simulink model "Q2_All"  (R2023b)
settings: Solver=VariableStepAuto  StartTime=0.0  StopTime=2000  RelTol=1e-3
libraries: simulink x17
settings Model: Creator=ArshiaGosh  LastModifiedBy=ArshiaGosh

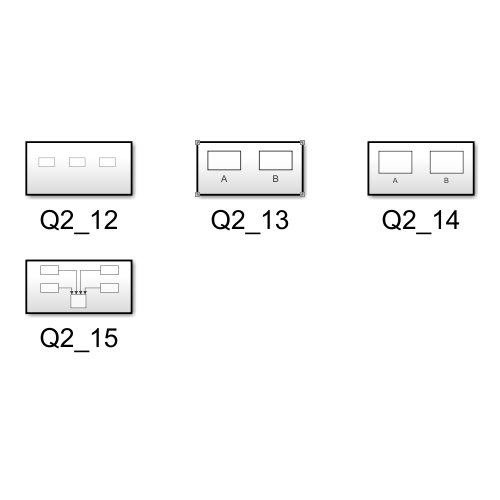
[thumbnail: Simulink's stored preview of the top-level diagram]
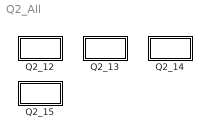
== system Q2_All ==
  Q2_12 : Subsystem
  Q2_13 : Subsystem
  Q2_14 : Subsystem
  Q2_15 : Subsystem

== system Q2_All/Q2_12 ==
  a) Step @ t=50 : Subsystem
  "b) Square Wave, T=100" : Subsystem
  c) Step @ t=50 a = -0.8 - 0.1sin(0.1t) b = 0.5 + ... : Subsystem

== system Q2_All/Q2_13 ==
  A : Subsystem
  B : Subsystem

== system Q2_All/Q2_14 ==
  A : Subsystem
  B : Subsystem

== system Q2_All/Q2_15 ==
  Scope : Scope  NumInputPorts=4
  landa=0.95 : Subsystem
  landa=0.99 : Subsystem
  landa=0.999 : Subsystem
  landa=1 : Subsystem
  wires:
  landa=1/1(thetak) -> Scope/1
  landa=0.99/1(thetak) -> Scope/3
  landa=0.999/1(thetak) -> Scope/2
  landa=0.95/1(thetak) -> Scope/4

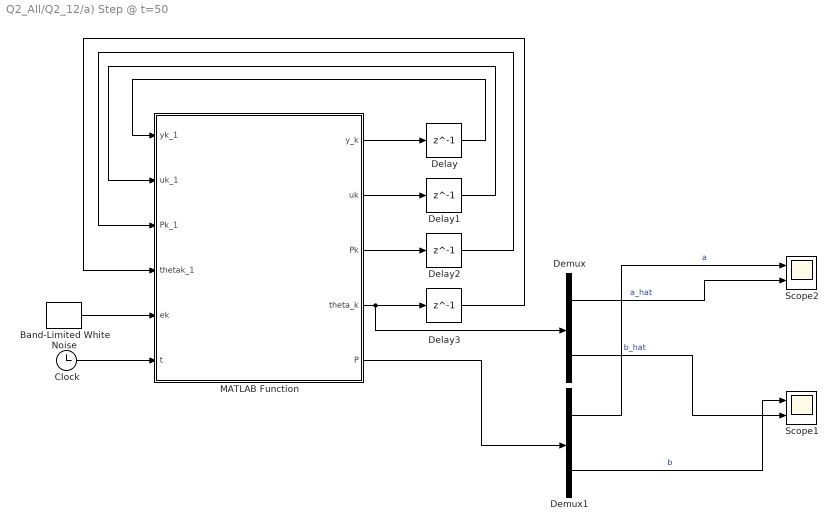
== system Q2_All/Q2_12/a) Step @ t=50 ==
  Band-Limited White Noise : simulink/Sources/Band-Limited White Noise  Cov=[0.5]  Ts=0.01  seed=[23341]
  Clock : Clock
  Delay : Delay  DelayLength=1  SampleTime=0.01
  Delay1 : Delay  DelayLength=1  SampleTime=0.01
  Delay2 : Delay  DelayLength=1  InitialCondition=100*eye(2,2)  SampleTime=0.01
  Delay3 : Delay  DelayLength=1  InitialCondition=[0;0]  SampleTime=0.01
  Demux : Demux  Outputs=2
  Demux1 : Demux  Outputs=2
  MATLAB Function : MATLAB Function  TreatAsAtomicUnit=on
  Scope1 : Scope  NumInputPorts=2
  Scope2 : Scope  NumInputPorts=2
  wires:
  Demux1/1 -> Scope2/1  "a"
  MATLAB Function/1(y_k) -> Delay/1
  MATLAB Function/5(P) -> Demux1/1
  Delay2/1 -> MATLAB Function/3(Pk_1)
  Clock/1 -> MATLAB Function/6(t)
  Demux/1 -> Scope2/2  "a_hat"
  Demux/2 -> Scope1/2  "b_hat"
  Delay3/1 -> MATLAB Function/4(thetak_1)
  MATLAB Function/4(theta_k) -> Demux/1, Delay3/1
  Band-Limited White Noise/1 -> MATLAB Function/5(ek)
  Delay/1 -> MATLAB Function/1(yk_1)
  MATLAB Function/3(Pk) -> Delay2/1
  MATLAB Function/2(uk) -> Delay1/1
  Delay1/1 -> MATLAB Function/2(uk_1)
  Demux1/2 -> Scope1/1  "b"

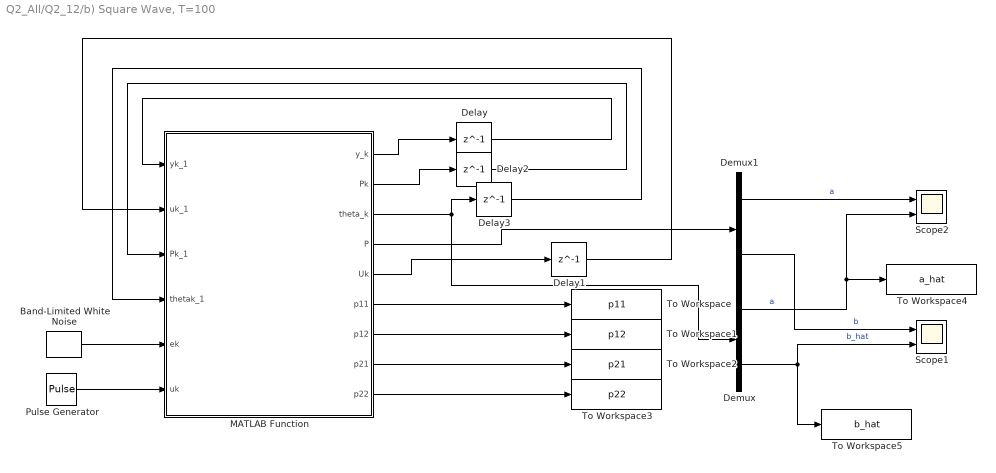
== system Q2_All/Q2_12/b) Square Wave, T=100 ==
  Band-Limited White Noise : simulink/Sources/Band-Limited White Noise  Cov=[0.5]  Ts=0.01  seed=[23341]
  Delay : Delay  DelayLength=1  SampleTime=0.01
  Delay1 : Delay  DelayLength=1  SampleTime=0.01
  Delay2 : Delay  DelayLength=1  InitialCondition=100*eye(2,2)  SampleTime=0.01
  Delay3 : Delay  DelayLength=1  InitialCondition=[0;0]  SampleTime=0.01
  Demux : Demux  Outputs=2
  Demux1 : Demux  Outputs=2
  MATLAB Function : MATLAB Function  TreatAsAtomicUnit=on
  Pulse Generator : DiscretePulseGenerator  PulseType=Time based  Period=100  PulseWidth=50
  Scope1 : Scope  NumInputPorts=2
  Scope2 : Scope  NumInputPorts=2
  To Workspace : ToWorkspace  VariableName=p11  SaveFormat=Timeseries  SampleTime=0.01
  To Workspace1 : ToWorkspace  VariableName=p12  SaveFormat=Timeseries  SampleTime=0.01
  To Workspace2 : ToWorkspace  VariableName=p21  SaveFormat=Timeseries  SampleTime=0.01
  To Workspace3 : ToWorkspace  VariableName=p22  SaveFormat=Timeseries  SampleTime=0.01
  To Workspace4 : ToWorkspace  VariableName=a_hat  SaveFormat=Timeseries  SampleTime=0.01
  To Workspace5 : ToWorkspace  VariableName=b_hat  SaveFormat=Timeseries  SampleTime=0.01
  wires:
  Demux1/2 -> Scope1/1  "b"
  Delay1/1 -> MATLAB Function/2(uk_1)
  MATLAB Function/2(Pk) -> Delay2/1
  Delay/1 -> MATLAB Function/1(yk_1)
  Band-Limited White Noise/1 -> MATLAB Function/5(ek)
  MATLAB Function/3(theta_k) -> Delay3/1, Demux/1
  Delay3/1 -> MATLAB Function/4(thetak_1)
  Demux/2 -> Scope1/2, To Workspace5/1  "b_hat"
  Delay2/1 -> MATLAB Function/3(Pk_1)
  MATLAB Function/4(P) -> Demux1/1
  MATLAB Function/1(y_k) -> Delay/1
  Demux1/1 -> Scope2/1  "a"
  Pulse Generator/1 -> MATLAB Function/6(uk)
  MATLAB Function/5(Uk) -> Delay1/1
  MATLAB Function/6(p11) -> To Workspace/1
  MATLAB Function/7(p12) -> To Workspace1/1
  MATLAB Function/8(p21) -> To Workspace2/1
  MATLAB Function/9(p22) -> To Workspace3/1
  Demux/1 -> To Workspace4/1, Scope2/2  "a"

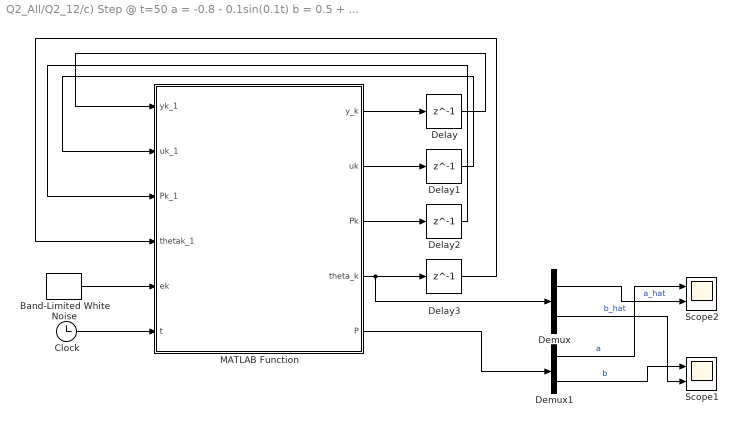
== system Q2_All/Q2_12/c) Step @ t=50 a = -0.8 - 0.1sin(0.1t) b = 0.5 + ... ==
  Band-Limited White Noise : simulink/Sources/Band-Limited White Noise  Cov=[0.5]  Ts=0.01  seed=[23341]
  Clock : Clock
  Delay : Delay  DelayLength=1  SampleTime=0.01
  Delay1 : Delay  DelayLength=1  SampleTime=0.01
  Delay2 : Delay  DelayLength=1  InitialCondition=100*eye(2,2)  SampleTime=0.01
  Delay3 : Delay  DelayLength=1  InitialCondition=[0;0]  SampleTime=0.01
  Demux : Demux  Outputs=2
  Demux1 : Demux  Outputs=2
  MATLAB Function : MATLAB Function  TreatAsAtomicUnit=on
  Scope1 : Scope  NumInputPorts=2
  Scope2 : Scope  NumInputPorts=2
  wires:
  Demux1/1 -> Scope2/1  "a"
  MATLAB Function/1(y_k) -> Delay/1
  MATLAB Function/5(P) -> Demux1/1
  Delay2/1 -> MATLAB Function/3(Pk_1)
  Clock/1 -> MATLAB Function/6(t)
  Demux/1 -> Scope2/2  "a_hat"
  Demux/2 -> Scope1/2  "b_hat"
  Delay3/1 -> MATLAB Function/4(thetak_1)
  MATLAB Function/4(theta_k) -> Demux/1, Delay3/1
  Band-Limited White Noise/1 -> MATLAB Function/5(ek)
  Delay/1 -> MATLAB Function/1(yk_1)
  MATLAB Function/3(Pk) -> Delay2/1
  MATLAB Function/2(uk) -> Delay1/1
  Delay1/1 -> MATLAB Function/2(uk_1)
  Demux1/2 -> Scope1/1  "b"

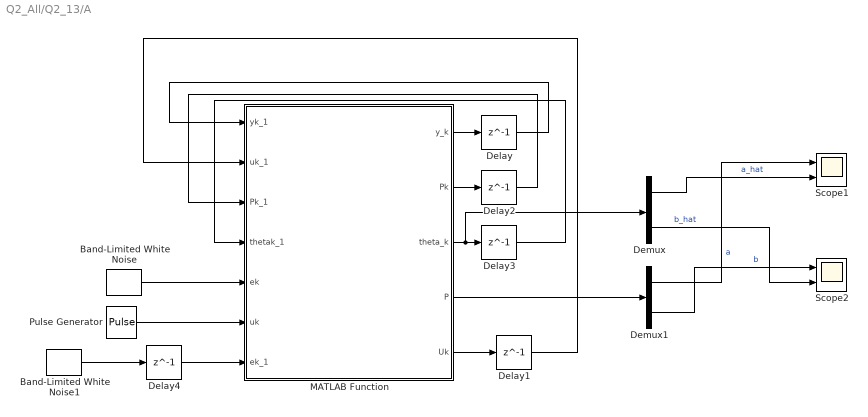
== system Q2_All/Q2_13/A ==
  Band-Limited White Noise : simulink/Sources/Band-Limited White Noise  Cov=[0.5]  Ts=0.01  seed=[23341]
  Band-Limited White Noise1 : simulink/Sources/Band-Limited White Noise  Cov=[0.5]  Ts=0.01  seed=[23341]
  Delay : Delay  DelayLength=1  SampleTime=0.01
  Delay1 : Delay  DelayLength=1  SampleTime=0.01
  Delay2 : Delay  DelayLength=1  InitialCondition=100*eye(2,2)  SampleTime=0.01
  Delay3 : Delay  DelayLength=1  InitialCondition=[0;0]  SampleTime=0.01
  Delay4 : Delay  DelayLength=1  SampleTime=0.01
  Demux : Demux  Outputs=2
  Demux1 : Demux  Outputs=2
  MATLAB Function : MATLAB Function  TreatAsAtomicUnit=on
  Pulse Generator : DiscretePulseGenerator  PulseType=Time based  Period=100  PulseWidth=50
  Scope1 : Scope  NumInputPorts=2
  Scope2 : Scope  NumInputPorts=2
  wires:
  Delay4/1 -> MATLAB Function/7(ek_1)
  Band-Limited White Noise1/1 -> Delay4/1
  MATLAB Function/5(Uk) -> Delay1/1
  Pulse Generator/1 -> MATLAB Function/6(uk)
  Demux1/1 -> Scope1/1  "a"
  MATLAB Function/1(y_k) -> Delay/1
  MATLAB Function/4(P) -> Demux1/1
  Delay2/1 -> MATLAB Function/3(Pk_1)
  Demux/1 -> Scope1/2  "a_hat"
  Demux/2 -> Scope2/2  "b_hat"
  Delay3/1 -> MATLAB Function/4(thetak_1)
  MATLAB Function/3(theta_k) -> Demux/1, Delay3/1
  Band-Limited White Noise/1 -> MATLAB Function/5(ek)
  Delay/1 -> MATLAB Function/1(yk_1)
  MATLAB Function/2(Pk) -> Delay2/1
  Delay1/1 -> MATLAB Function/2(uk_1)
  Demux1/2 -> Scope2/1  "b"

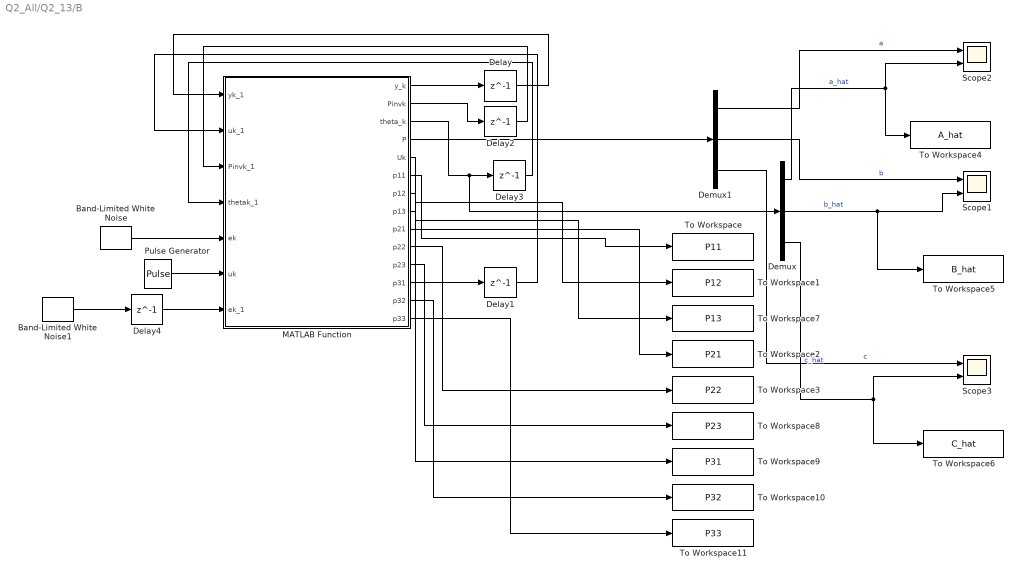
== system Q2_All/Q2_13/B ==
  Band-Limited White Noise : simulink/Sources/Band-Limited White Noise  Cov=[0.5]  Ts=0.01  seed=[23341]
  Band-Limited White Noise1 : simulink/Sources/Band-Limited White Noise  Cov=[0.5]  Ts=0.01  seed=[23341]
  Delay : Delay  DelayLength=1  SampleTime=0.01
  Delay1 : Delay  DelayLength=1  SampleTime=0.01
  Delay2 : Delay  DelayLength=1  InitialCondition=100*eye(3,3)  SampleTime=0.01
  Delay3 : Delay  DelayLength=1  InitialCondition=[0;0;0]  SampleTime=0.01
  Delay4 : Delay  DelayLength=1  SampleTime=0.01
  Demux : Demux  Outputs=3
  Demux1 : Demux  Outputs=3
  MATLAB Function : MATLAB Function  TreatAsAtomicUnit=on
  Pulse Generator : DiscretePulseGenerator  PulseType=Time based  Period=100  PulseWidth=50
  Scope1 : Scope  NumInputPorts=2
  Scope2 : Scope  NumInputPorts=2
  Scope3 : Scope  NumInputPorts=2
  To Workspace : ToWorkspace  VariableName=P11  SaveFormat=Timeseries  SampleTime=0.01
  To Workspace1 : ToWorkspace  VariableName=P12  SaveFormat=Timeseries  SampleTime=0.01
  To Workspace10 : ToWorkspace  VariableName=P32  SaveFormat=Timeseries  SampleTime=0.01
  To Workspace11 : ToWorkspace  VariableName=P33  SaveFormat=Timeseries  SampleTime=0.01
  To Workspace2 : ToWorkspace  VariableName=P21  SaveFormat=Timeseries  SampleTime=0.01
  To Workspace3 : ToWorkspace  VariableName=P22  SaveFormat=Timeseries  SampleTime=0.01
  To Workspace4 : ToWorkspace  VariableName=A_hat  SaveFormat=Timeseries  SampleTime=-1
  To Workspace5 : ToWorkspace  VariableName=B_hat  SaveFormat=Timeseries  SampleTime=-1
  To Workspace6 : ToWorkspace  VariableName=C_hat  SaveFormat=Timeseries  SampleTime=-1
  To Workspace7 : ToWorkspace  VariableName=P13  SaveFormat=Timeseries  SampleTime=0.01
  To Workspace8 : ToWorkspace  VariableName=P23  SaveFormat=Timeseries  SampleTime=0.01
  To Workspace9 : ToWorkspace  VariableName=P31  SaveFormat=Timeseries  SampleTime=0.01
  wires:
  Demux1/2 -> Scope1/1  "b"
  Delay1/1 -> MATLAB Function/2(uk_1)
  MATLAB Function/2(Pinvk) -> Delay2/1
  Delay/1 -> MATLAB Function/1(yk_1)
  Band-Limited White Noise/1 -> MATLAB Function/5(ek)
  MATLAB Function/3(theta_k) -> Demux/1, Delay3/1
  Delay3/1 -> MATLAB Function/4(thetak_1)
  Demux/2 -> Scope1/2, To Workspace5/1  "b_hat"
  Demux/1 -> Scope2/2, To Workspace4/1  "a_hat"
  Delay2/1 -> MATLAB Function/3(Pinvk_1)
  MATLAB Function/4(P) -> Demux1/1
  MATLAB Function/1(y_k) -> Delay/1
  Demux1/1 -> Scope2/1  "a"
  Pulse Generator/1 -> MATLAB Function/6(uk)
  MATLAB Function/5(Uk) -> Delay1/1
  Band-Limited White Noise1/1 -> Delay4/1
  Delay4/1 -> MATLAB Function/7(ek_1)
  Demux1/3 -> Scope3/1  "c"
  Demux/3 -> Scope3/2, To Workspace6/1  "c_hat"
  MATLAB Function/6(p11) -> To Workspace/1
  MATLAB Function/7(p12) -> To Workspace1/1
  MATLAB Function/9(p21) -> To Workspace2/1
  MATLAB Function/10(p22) -> To Workspace3/1
  MATLAB Function/8(p13) -> To Workspace7/1
  MATLAB Function/11(p23) -> To Workspace8/1
  MATLAB Function/12(p31) -> To Workspace9/1
  MATLAB Function/13(p32) -> To Workspace10/1
  MATLAB Function/14(p33) -> To Workspace11/1

== system Q2_All/Q2_14/A ==
  u(k)=-0.2y(k) : Subsystem
  u(k)=-0.32y(k_1) : Subsystem

== system Q2_All/Q2_14/B ==
  landa=0.95 : Subsystem
  landa=0.99 : Subsystem
  landa=0.999 : Subsystem
  landa=1 : Subsystem

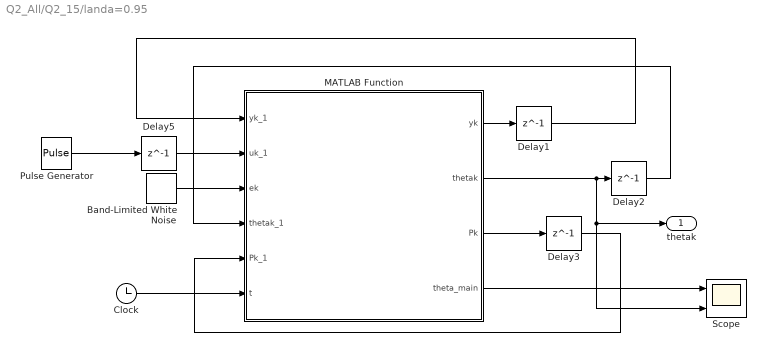
== system Q2_All/Q2_15/landa=0.95 ==
  Band-Limited White Noise : simulink/Sources/Band-Limited White Noise  Cov=[0.5]  Ts=1  seed=[23341]
  Clock : Clock
  Delay1 : Delay  DelayLength=1  SampleTime=1
  Delay2 : Delay  DelayLength=1  InitialCondition=[0;0]  SampleTime=1
  Delay3 : Delay  DelayLength=1  InitialCondition=100*eye(2,2)  SampleTime=1
  Delay5 : Delay  DelayLength=1  SampleTime=1
  MATLAB Function : MATLAB Function  TreatAsAtomicUnit=on
  Pulse Generator : DiscretePulseGenerator  PulseType=Time based  Period=100  PulseWidth=50
  Scope : Scope  NumInputPorts=2
  thetak : Outport
  wires:
  Clock/1 -> MATLAB Function/6(t)
  MATLAB Function/3(Pk) -> Delay3/1
  Band-Limited White Noise/1 -> MATLAB Function/3(ek)
  Pulse Generator/1 -> Delay5/1
  Delay5/1 -> MATLAB Function/2(uk_1)
  Delay3/1 -> MATLAB Function/5(Pk_1)
  MATLAB Function/4(theta_main) -> Scope/1
  MATLAB Function/1(yk) -> Delay1/1
  Delay1/1 -> MATLAB Function/1(yk_1)
  Delay2/1 -> MATLAB Function/4(thetak_1)
  MATLAB Function/2(thetak) -> thetak/1, Scope/2, Delay2/1

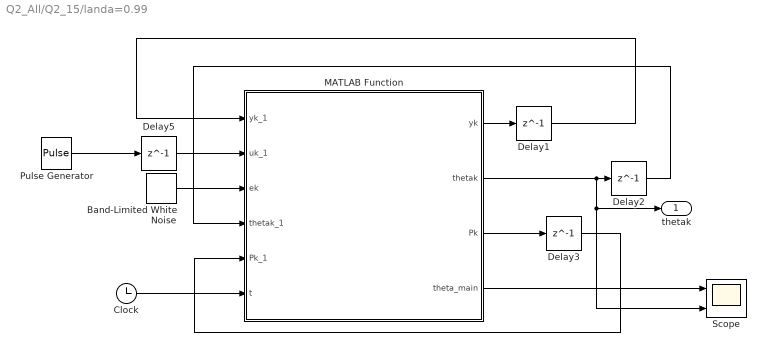
== system Q2_All/Q2_15/landa=0.99 ==
  Band-Limited White Noise : simulink/Sources/Band-Limited White Noise  Cov=[0.5]  Ts=1  seed=[23341]
  Clock : Clock
  Delay1 : Delay  DelayLength=1  SampleTime=1
  Delay2 : Delay  DelayLength=1  InitialCondition=[0;0]  SampleTime=1
  Delay3 : Delay  DelayLength=1  InitialCondition=100*eye(2,2)  SampleTime=1
  Delay5 : Delay  DelayLength=1  SampleTime=1
  MATLAB Function : MATLAB Function  TreatAsAtomicUnit=on
  Pulse Generator : DiscretePulseGenerator  PulseType=Time based  Period=100  PulseWidth=50
  Scope : Scope  NumInputPorts=2
  thetak : Outport
  wires:
  Clock/1 -> MATLAB Function/6(t)
  MATLAB Function/3(Pk) -> Delay3/1
  Band-Limited White Noise/1 -> MATLAB Function/3(ek)
  Pulse Generator/1 -> Delay5/1
  Delay5/1 -> MATLAB Function/2(uk_1)
  Delay3/1 -> MATLAB Function/5(Pk_1)
  MATLAB Function/4(theta_main) -> Scope/1
  MATLAB Function/1(yk) -> Delay1/1
  Delay1/1 -> MATLAB Function/1(yk_1)
  Delay2/1 -> MATLAB Function/4(thetak_1)
  MATLAB Function/2(thetak) -> thetak/1, Scope/2, Delay2/1

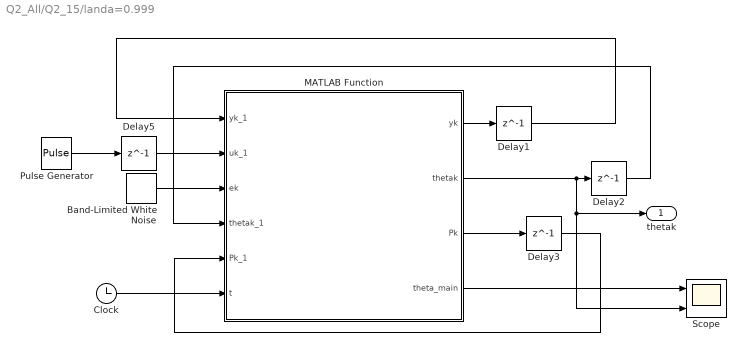
== system Q2_All/Q2_15/landa=0.999 ==
  Band-Limited White Noise : simulink/Sources/Band-Limited White Noise  Cov=[0.5]  Ts=1  seed=[23341]
  Clock : Clock
  Delay1 : Delay  DelayLength=1  SampleTime=1
  Delay2 : Delay  DelayLength=1  InitialCondition=[0;0]  SampleTime=1
  Delay3 : Delay  DelayLength=1  InitialCondition=100*eye(2,2)  SampleTime=1
  Delay5 : Delay  DelayLength=1  SampleTime=1
  MATLAB Function : MATLAB Function  TreatAsAtomicUnit=on
  Pulse Generator : DiscretePulseGenerator  PulseType=Time based  Period=100  PulseWidth=50
  Scope : Scope  NumInputPorts=2
  thetak : Outport
  wires:
  Clock/1 -> MATLAB Function/6(t)
  MATLAB Function/3(Pk) -> Delay3/1
  Band-Limited White Noise/1 -> MATLAB Function/3(ek)
  Pulse Generator/1 -> Delay5/1
  Delay5/1 -> MATLAB Function/2(uk_1)
  Delay3/1 -> MATLAB Function/5(Pk_1)
  MATLAB Function/4(theta_main) -> Scope/1
  MATLAB Function/1(yk) -> Delay1/1
  Delay1/1 -> MATLAB Function/1(yk_1)
  Delay2/1 -> MATLAB Function/4(thetak_1)
  MATLAB Function/2(thetak) -> thetak/1, Scope/2, Delay2/1

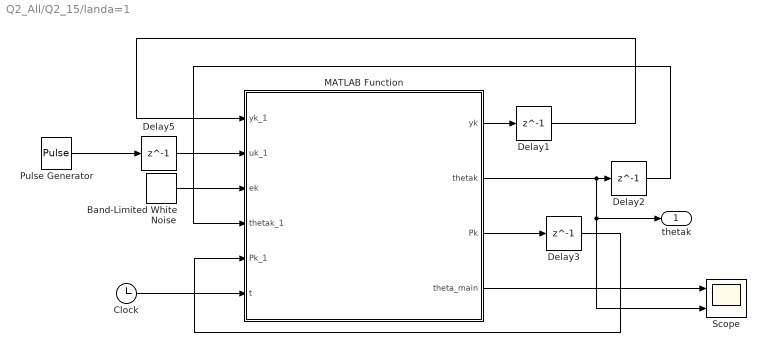
== system Q2_All/Q2_15/landa=1 ==
  Band-Limited White Noise : simulink/Sources/Band-Limited White Noise  Cov=[0.5]  Ts=1  seed=[23341]
  Clock : Clock
  Delay1 : Delay  DelayLength=1  SampleTime=1
  Delay2 : Delay  DelayLength=1  InitialCondition=[0;0]  SampleTime=1
  Delay3 : Delay  DelayLength=1  InitialCondition=100*eye(2,2)  SampleTime=1
  Delay5 : Delay  DelayLength=1  SampleTime=1
  MATLAB Function : MATLAB Function  TreatAsAtomicUnit=on
  Pulse Generator : DiscretePulseGenerator  PulseType=Time based  Period=100  PulseWidth=50
  Scope : Scope  NumInputPorts=2
  thetak : Outport
  wires:
  Clock/1 -> MATLAB Function/6(t)
  MATLAB Function/1(yk) -> Delay1/1
  MATLAB Function/3(Pk) -> Delay3/1
  Delay1/1 -> MATLAB Function/1(yk_1)
  Band-Limited White Noise/1 -> MATLAB Function/3(ek)
  Delay2/1 -> MATLAB Function/4(thetak_1)
  Delay3/1 -> MATLAB Function/5(Pk_1)
  Delay5/1 -> MATLAB Function/2(uk_1)
  Pulse Generator/1 -> Delay5/1
  MATLAB Function/4(theta_main) -> Scope/1
  MATLAB Function/2(thetak) -> thetak/1, Scope/2, Delay2/1

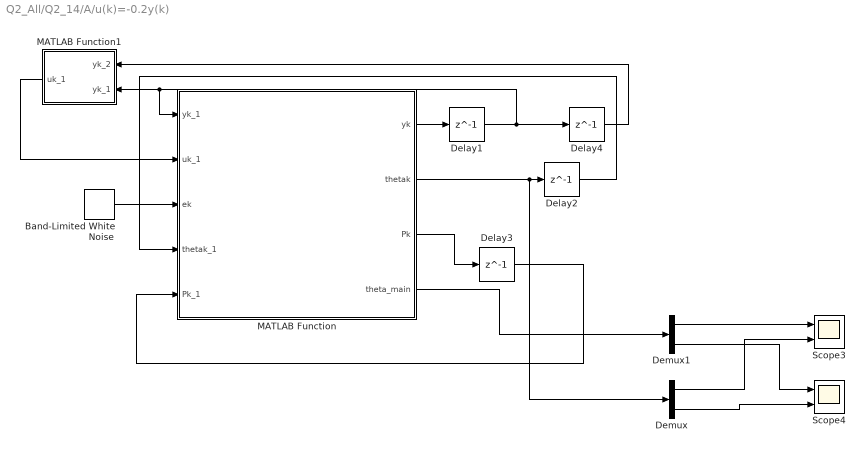
== system Q2_All/Q2_14/A/u(k)=-0.2y(k) ==
  Band-Limited White Noise : simulink/Sources/Band-Limited White Noise  Cov=[0.5]  Ts=0.01  seed=[23341]
  Delay1 : Delay  DelayLength=1  SampleTime=0.01
  Delay2 : Delay  DelayLength=1  InitialCondition=[0;0]  SampleTime=0.01
  Delay3 : Delay  DelayLength=1  InitialCondition=.01*eye(2,2)  SampleTime=0.01
  Delay4 : Delay  DelayLength=1  SampleTime=0.01
  Demux : Demux  Outputs=2
  Demux1 : Demux  Outputs=2
  MATLAB Function : MATLAB Function  TreatAsAtomicUnit=on
  MATLAB Function1 : MATLAB Function  TreatAsAtomicUnit=on
  Scope3 : Scope  NumInputPorts=2
  Scope4 : Scope  NumInputPorts=2
  wires:
  MATLAB Function/3(Pk) -> Delay3/1
  Band-Limited White Noise/1 -> MATLAB Function/3(ek)
  MATLAB Function/1(yk) -> Delay1/1
  Delay3/1 -> MATLAB Function/5(Pk_1)
  Delay2/1 -> MATLAB Function/4(thetak_1)
  Demux1/2 -> Scope4/1
  Demux/1 -> Scope3/2
  MATLAB Function/2(thetak) -> Demux/1, Delay2/1
  Demux/2 -> Scope4/2
  Demux1/1 -> Scope3/1
  MATLAB Function1/1(uk_1) -> MATLAB Function/2(uk_1)
  MATLAB Function/4(theta_main) -> Demux1/1
  Delay4/1 -> MATLAB Function1/1(yk_2)
  Delay1/1 -> Delay4/1, MATLAB Function1/2(yk_1), MATLAB Function/1(yk_1)

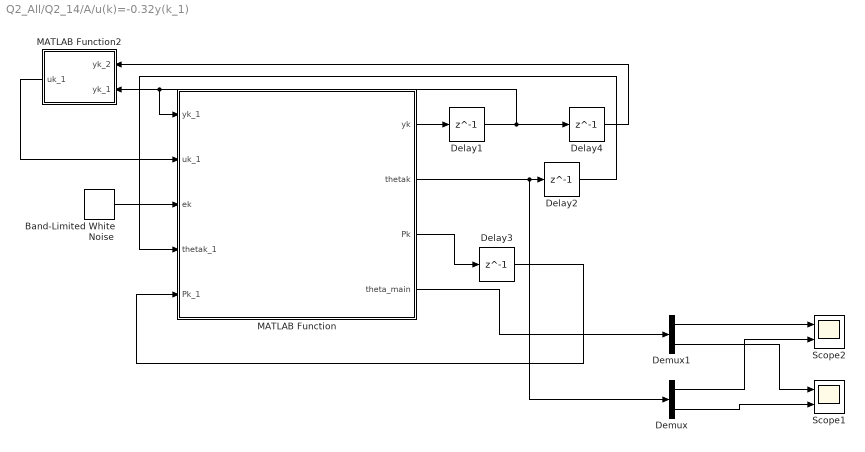
== system Q2_All/Q2_14/A/u(k)=-0.32y(k_1) ==
  Band-Limited White Noise : simulink/Sources/Band-Limited White Noise  Cov=[0.5]  Ts=0.01  seed=[23341]
  Delay1 : Delay  DelayLength=1  SampleTime=0.01
  Delay2 : Delay  DelayLength=1  InitialCondition=[0;0]  SampleTime=0.01
  Delay3 : Delay  DelayLength=1  InitialCondition=.01*eye(2,2)  SampleTime=0.01
  Delay4 : Delay  DelayLength=1  SampleTime=0.01
  Demux : Demux  Outputs=2
  Demux1 : Demux  Outputs=2
  MATLAB Function : MATLAB Function  TreatAsAtomicUnit=on
  MATLAB Function2 : MATLAB Function  TreatAsAtomicUnit=on
  Scope1 : Scope  NumInputPorts=2
  Scope2 : Scope  NumInputPorts=2
  wires:
  MATLAB Function/4(theta_main) -> Demux1/1
  Delay4/1 -> MATLAB Function2/1(yk_2)
  MATLAB Function2/1(uk_1) -> MATLAB Function/2(uk_1)
  Delay2/1 -> MATLAB Function/4(thetak_1)
  Delay3/1 -> MATLAB Function/5(Pk_1)
  MATLAB Function/1(yk) -> Delay1/1
  Demux1/2 -> Scope1/1
  Delay1/1 -> Delay4/1, MATLAB Function2/2(yk_1), MATLAB Function/1(yk_1)
  Demux1/1 -> Scope2/1
  Demux/2 -> Scope1/2
  Demux/1 -> Scope2/2
  MATLAB Function/3(Pk) -> Delay3/1
  MATLAB Function/2(thetak) -> Demux/1, Delay2/1
  Band-Limited White Noise/1 -> MATLAB Function/3(ek)

== system Q2_All/Q2_14/B/landa=0.95 ==
  Band-Limited White Noise : simulink/Sources/Band-Limited White Noise  Cov=[0.5]  Ts=1  seed=[23341]
  Clock : Clock
  Delay1 : Delay  DelayLength=1  SampleTime=1
  Delay2 : Delay  DelayLength=1  InitialCondition=[0;0]  SampleTime=1
  Delay3 : Delay  DelayLength=1  InitialCondition=100*eye(2,2)  SampleTime=1
  Delay5 : Delay  DelayLength=1  SampleTime=1
  MATLAB Function : MATLAB Function  TreatAsAtomicUnit=on
  Pulse Generator : DiscretePulseGenerator  PulseType=Time based  Period=100  PulseWidth=50
  Scope : Scope  NumInputPorts=2
  wires:
  Clock/1 -> MATLAB Function/6(t)
  MATLAB Function/3(Pk) -> Delay3/1
  Band-Limited White Noise/1 -> MATLAB Function/3(ek)
  Pulse Generator/1 -> Delay5/1
  Delay5/1 -> MATLAB Function/2(uk_1)
  Delay3/1 -> MATLAB Function/5(Pk_1)
  MATLAB Function/4(theta_main) -> Scope/1
  MATLAB Function/1(yk) -> Delay1/1
  Delay1/1 -> MATLAB Function/1(yk_1)
  Delay2/1 -> MATLAB Function/4(thetak_1)
  MATLAB Function/2(thetak) -> Scope/2, Delay2/1

== system Q2_All/Q2_14/B/landa=0.99 ==
  Band-Limited White Noise : simulink/Sources/Band-Limited White Noise  Cov=[0.5]  Ts=1  seed=[23341]
  Clock : Clock
  Delay1 : Delay  DelayLength=1  SampleTime=1
  Delay2 : Delay  DelayLength=1  InitialCondition=[0;0]  SampleTime=1
  Delay3 : Delay  DelayLength=1  InitialCondition=100*eye(2,2)  SampleTime=1
  Delay5 : Delay  DelayLength=1  SampleTime=1
  MATLAB Function : MATLAB Function  TreatAsAtomicUnit=on
  Pulse Generator : DiscretePulseGenerator  PulseType=Time based  Period=100  PulseWidth=50
  Scope : Scope  NumInputPorts=2
  wires:
  Clock/1 -> MATLAB Function/6(t)
  MATLAB Function/3(Pk) -> Delay3/1
  Band-Limited White Noise/1 -> MATLAB Function/3(ek)
  Pulse Generator/1 -> Delay5/1
  Delay5/1 -> MATLAB Function/2(uk_1)
  Delay3/1 -> MATLAB Function/5(Pk_1)
  MATLAB Function/4(theta_main) -> Scope/1
  MATLAB Function/1(yk) -> Delay1/1
  Delay1/1 -> MATLAB Function/1(yk_1)
  Delay2/1 -> MATLAB Function/4(thetak_1)
  MATLAB Function/2(thetak) -> Scope/2, Delay2/1

== system Q2_All/Q2_14/B/landa=0.999 ==
  Band-Limited White Noise : simulink/Sources/Band-Limited White Noise  Cov=[0.5]  Ts=1  seed=[23341]
  Clock : Clock
  Delay1 : Delay  DelayLength=1  SampleTime=1
  Delay2 : Delay  DelayLength=1  InitialCondition=[0;0]  SampleTime=1
  Delay3 : Delay  DelayLength=1  InitialCondition=100*eye(2,2)  SampleTime=1
  Delay5 : Delay  DelayLength=1  SampleTime=1
  MATLAB Function : MATLAB Function  TreatAsAtomicUnit=on
  Pulse Generator : DiscretePulseGenerator  PulseType=Time based  Period=100  PulseWidth=50
  Scope : Scope  NumInputPorts=2
  wires:
  Clock/1 -> MATLAB Function/6(t)
  MATLAB Function/3(Pk) -> Delay3/1
  Band-Limited White Noise/1 -> MATLAB Function/3(ek)
  Pulse Generator/1 -> Delay5/1
  Delay5/1 -> MATLAB Function/2(uk_1)
  Delay3/1 -> MATLAB Function/5(Pk_1)
  MATLAB Function/4(theta_main) -> Scope/1
  MATLAB Function/1(yk) -> Delay1/1
  Delay1/1 -> MATLAB Function/1(yk_1)
  Delay2/1 -> MATLAB Function/4(thetak_1)
  MATLAB Function/2(thetak) -> Scope/2, Delay2/1

== system Q2_All/Q2_14/B/landa=1 ==
  Band-Limited White Noise : simulink/Sources/Band-Limited White Noise  Cov=[0.5]  Ts=1  seed=[23341]
  Clock : Clock
  Delay1 : Delay  DelayLength=1  SampleTime=1
  Delay2 : Delay  DelayLength=1  InitialCondition=[0;0]  SampleTime=1
  Delay3 : Delay  DelayLength=1  InitialCondition=100*eye(2,2)  SampleTime=1
  Delay5 : Delay  DelayLength=1  SampleTime=1
  MATLAB Function : MATLAB Function  TreatAsAtomicUnit=on
  Pulse Generator : DiscretePulseGenerator  PulseType=Time based  Period=100  PulseWidth=50
  Scope : Scope  NumInputPorts=2
  wires:
  Clock/1 -> MATLAB Function/6(t)
  MATLAB Function/1(yk) -> Delay1/1
  MATLAB Function/3(Pk) -> Delay3/1
  Delay1/1 -> MATLAB Function/1(yk_1)
  Band-Limited White Noise/1 -> MATLAB Function/3(ek)
  Delay2/1 -> MATLAB Function/4(thetak_1)
  Delay3/1 -> MATLAB Function/5(Pk_1)
  Delay5/1 -> MATLAB Function/2(uk_1)
  Pulse Generator/1 -> Delay5/1
  MATLAB Function/4(theta_main) -> Scope/1
  MATLAB Function/2(thetak) -> Scope/2, Delay2/1

== matlab function Q2_All/Q2_13/A/MATLAB Function ==
  data: yk_1 input; y_k output; uk_1 input; Pk_1 input; thetak_1 input; ek input; Pk output; theta_k output; P output; uk input; Uk output; ek_1 input
function [y_k,Pk,theta_k,P,Uk] = fcn(yk_1,uk_1,Pk_1,thetak_1,ek,uk,ek_1)
a=-0.8;
b=0.5;
c=-0.5;
P=[a;b];
Uk=uk;

sik=[-yk_1 uk_1]';
y_k=-a*yk_1+b*uk_1+ek+c*ek_1;

Kk=Pk_1*sik*pinv(1+sik'*Pk_1*sik);
Pk=(eye(2,2)-Kk*sik')*Pk_1;
theta_k=thetak_1+Kk*(y_k-sik'*thetak_1);

== matlab function Q2_All/Q2_14/A/u(k)=-0.2y(k)/MATLAB Function ==
  data: yk_1 input; yk output; uk_1 input; ek input; thetak_1 input; Pk_1 input; thetak output; Pk output; theta_main output
function [yk,thetak,Pk,theta_main] = fcn(yk_1,uk_1,ek,thetak_1,Pk_1)
a=-0.8;
b=0.5;
theta_main=[a;b];
%model dynamic
yk=-a*yk_1+b*uk_1+ek;
%estimate
phi=[-yk_1;uk_1];
Kk=Pk_1*phi*pinv(1+phi'*Pk_1*phi);
Pk=(eye(2,2)-Kk*phi')*Pk_1;
thetak=thetak_1+Kk*(yk-phi'*thetak_1);

== matlab function Q2_All/Q2_14/A/u(k)=-0.2y(k)/MATLAB Function1 ==
  data: yk_2 input; uk_1 output; yk_1 input
function uk_1   = fcn(yk_2,yk_1)
uk_1=-0.2*(yk_1);
%  uk_1=-0.2*yk_2;

== matlab function Q2_All/Q2_14/A/u(k)=-0.32y(k_1)/MATLAB Function ==
  data: yk_1 input; yk output; uk_1 input; ek input; thetak_1 input; Pk_1 input; thetak output; Pk output; theta_main output
function [yk,thetak,Pk,theta_main] = fcn(yk_1,uk_1,ek,thetak_1,Pk_1)
a=-0.8;
b=0.5;
theta_main=[a;b];
%model dynamic
yk=-a*yk_1+b*uk_1+ek;
%estimate
phi=[-yk_1;uk_1];
Kk=Pk_1*phi*pinv(1+phi'*Pk_1*phi);
Pk=(eye(2,2)-Kk*phi')*Pk_1;
thetak=thetak_1+Kk*(yk-phi'*thetak_1);

== matlab function Q2_All/Q2_14/B/landa=0.999/MATLAB Function ==
  data: yk_1 input; yk output; uk_1 input; ek input; thetak_1 input; Pk_1 input; thetak output; Pk output; theta_main output; t input
function [yk,thetak,Pk,theta_main] = fcn(yk_1,uk_1,ek,thetak_1,Pk_1,t)
b=0.5;
a=-0.8;
landa=0.999;

% if t>0 && t<=500
%     a=-0.8;
% else
%     a=0.8;
% end
theta_main=[a;b];
%model dynamic
yk=-a*yk_1+b*uk_1+ek;
%estimate
phi=[-yk_1;uk_1];
Kk=Pk_1*phi*pinv(landa*1+phi'*Pk_1*phi);
Pk=(eye(2,2)-Kk*phi')*Pk_1/landa;
thetak=thetak_1+Kk*(yk-phi'*thetak_1);

== matlab function Q2_All/Q2_14/B/landa=0.95/MATLAB Function ==
  data: yk_1 input; yk output; uk_1 input; ek input; thetak_1 input; Pk_1 input; thetak output; Pk output; theta_main output; t input
function [yk,thetak,Pk,theta_main] = fcn(yk_1,uk_1,ek,thetak_1,Pk_1,t)
b=0.5;
a=-0.8;
landa=0.95;

% if t>0 && t<=500
%     a=-0.8;
% else
%     a=0.8;
% end
theta_main=[a;b];
%model dynamic
yk=-a*yk_1+b*uk_1+ek;
%estimate
phi=[-yk_1;uk_1];
Kk=Pk_1*phi*pinv(landa*1+phi'*Pk_1*phi);
Pk=(eye(2,2)-Kk*phi')*Pk_1/landa;
thetak=thetak_1+Kk*(yk-phi'*thetak_1);

== matlab function Q2_All/Q2_14/B/landa=0.99/MATLAB Function ==
  data: yk_1 input; yk output; uk_1 input; ek input; thetak_1 input; Pk_1 input; thetak output; Pk output; theta_main output; t input
function [yk,thetak,Pk,theta_main] = fcn(yk_1,uk_1,ek,thetak_1,Pk_1,t)
b=0.5;
a=-0.8;
landa=0.99;

% if t>0 && t<=500
%     a=-0.8;
% else
%     a=0.8;
% end
theta_main=[a;b];
%model dynamic
yk=-a*yk_1+b*uk_1+ek;
%estimate
phi=[-yk_1;uk_1];
Kk=Pk_1*phi*pinv(landa*1+phi'*Pk_1*phi);
Pk=(eye(2,2)-Kk*phi')*Pk_1/landa;
thetak=thetak_1+Kk*(yk-phi'*thetak_1);

== matlab function Q2_All/Q2_15/landa=0.95/MATLAB Function ==
  data: yk_1 input; yk output; uk_1 input; ek input; thetak_1 input; Pk_1 input; thetak output; Pk output; theta_main output; t input
function [yk,thetak,Pk,theta_main] = fcn(yk_1,uk_1,ek,thetak_1,Pk_1,t)
b=0.5;
a=-0.8;
landa=0.95;

% if t>0 && t<=500
%     a=-0.8;
% else
%     a=0.8;
% end
theta_main=[a;b];
%model dynamic
yk=-a*yk_1+b*uk_1+ek;
%estimate
phi=[-yk_1;uk_1];
Kk=Pk_1*phi*pinv(landa*1+phi'*Pk_1*phi);
Pk=(eye(2,2)-Kk*phi')*Pk_1/landa;
thetak=thetak_1+Kk*(yk-phi'*thetak_1);

== matlab function Q2_All/Q2_14/B/landa=1/MATLAB Function ==
  data: yk_1 input; yk output; uk_1 input; ek input; thetak_1 input; Pk_1 input; thetak output; Pk output; theta_main output; t input
function [yk,thetak,Pk,theta_main] = fcn(yk_1,uk_1,ek,thetak_1,Pk_1,t)
b=0.5;
a=-0.8;
landa=1;

% if t>0 && t<=500
%     a=-0.8;
% else
%     a=0.8;
% end
theta_main=[a;b];
%model dynamic
yk=-a*yk_1+b*uk_1+ek;
%estimate
phi=[-yk_1;uk_1];
Kk=Pk_1*phi*pinv(landa*1+phi'*Pk_1*phi);
Pk=(eye(2,2)-Kk*phi')*Pk_1/landa;
thetak=thetak_1+Kk*(yk-phi'*thetak_1);

== matlab function Q2_All/Q2_14/A/u(k)=-0.32y(k_1)/MATLAB Function2 ==
  data: yk_2 input; uk_1 output; yk_1 input
function uk_1   = fcn(yk_2,yk_1)
uk_1=-0.32*(yk_2);
%  uk_1=-0.2*yk_2;

== matlab function Q2_All/Q2_15/landa=0.99/MATLAB Function ==
  data: yk_1 input; yk output; uk_1 input; ek input; thetak_1 input; Pk_1 input; thetak output; Pk output; theta_main output; t input
function [yk,thetak,Pk,theta_main] = fcn(yk_1,uk_1,ek,thetak_1,Pk_1,t)
b=0.5;
a=-0.8;
landa=0.99;

% if t>0 && t<=500
%     a=-0.8;
% else
%     a=0.8;
% end
theta_main=[a;b];
%model dynamic
yk=-a*yk_1+b*uk_1+ek;
%estimate
phi=[-yk_1;uk_1];
Kk=Pk_1*phi*pinv(landa*1+phi'*Pk_1*phi);
Pk=(eye(2,2)-Kk*phi')*Pk_1/landa;
thetak=thetak_1+Kk*(yk-phi'*thetak_1);

== matlab function Q2_All/Q2_15/landa=0.999/MATLAB Function ==
  data: yk_1 input; yk output; uk_1 input; ek input; thetak_1 input; Pk_1 input; thetak output; Pk output; theta_main output; t input
function [yk,thetak,Pk,theta_main] = fcn(yk_1,uk_1,ek,thetak_1,Pk_1,t)
b=0.5;
a=-0.8;
landa=0.999;

% if t>0 && t<=500
%     a=-0.8;
% else
%     a=0.8;
% end
theta_main=[a;b];
%model dynamic
yk=-a*yk_1+b*uk_1+ek;
%estimate
phi=[-yk_1;uk_1];
Kk=Pk_1*phi*pinv(landa*1+phi'*Pk_1*phi);
Pk=(eye(2,2)-Kk*phi')*Pk_1/landa;
thetak=thetak_1+Kk*(yk-phi'*thetak_1);

== matlab function Q2_All/Q2_15/landa=1/MATLAB Function ==
  data: yk_1 input; yk output; uk_1 input; ek input; thetak_1 input; Pk_1 input; thetak output; Pk output; theta_main output; t input
function [yk,thetak,Pk,theta_main] = fcn(yk_1,uk_1,ek,thetak_1,Pk_1,t)
b=0.5;
a=-0.8;
landa=1;

% if t>0 && t<=500
%     a=-0.8;
% else
%     a=0.8;
% end
theta_main=[a;b];
%model dynamic
yk=-a*yk_1+b*uk_1+ek;
%estimate
phi=[-yk_1;uk_1];
Kk=Pk_1*phi*pinv(landa*1+phi'*Pk_1*phi);
Pk=(eye(2,2)-Kk*phi')*Pk_1/landa;
thetak=thetak_1+Kk*(yk-phi'*thetak_1);

== matlab function Q2_All/Q2_12/b) Square Wave, T=100/MATLAB Function ==
  data: yk_1 input; y_k output; uk_1 input; Pk_1 input; thetak_1 input; ek input; Pk output; theta_k output; P output; uk input; Uk output; p11 output; p12 output; p21 output; p22 output
function [y_k,Pk,theta_k,P,Uk,p11,p12,p21, p22] = fcn(yk_1,uk_1,Pk_1,thetak_1,ek,uk)
a=-0.8;
b=0.5;
P=[a;b];
Uk=uk;

sik=[-yk_1 uk_1]';
y_k=-a*yk_1+b*uk_1+ek;

Kk=Pk_1*sik*pinv(1+sik'*Pk_1*sik);
Pk=(eye(2,2)-Kk*sik')*Pk_1;
theta_k=thetak_1+Kk*(y_k-sik'*thetak_1);
p11=Pk(1,1);
p12=Pk(1,2);
p21=Pk(2,1);
p22=Pk(2,2);

== matlab function Q2_All/Q2_12/a) Step @ t=50/MATLAB Function ==
  data: yk_1 input; y_k output; uk_1 input; Pk_1 input; thetak_1 input; ek input; uk output; Pk output; theta_k output; t input; P output
function [y_k,uk,Pk,theta_k,P] = fcn(yk_1,uk_1,Pk_1,thetak_1,ek,t)
a=-0.8;
b=0.5;
P=[a;b];

if t>=0 && t<=50
    uk=0;
elseif t>=50 && t<51
    uk=1;
else
    uk=0;
end

sik=[-yk_1 uk_1]';
y_k=-a*yk_1+b*uk_1+ek;

Kk=Pk_1*sik*pinv(1+sik'*Pk_1*sik);
Pk=(eye(2,2)-Kk*sik')*Pk_1;
theta_k=thetak_1+Kk*(y_k-sik'*thetak_1);

== matlab function Q2_All/Q2_12/c) Step @ t=50 a = -0.8 - 0.1sin(0.1t) b = 0.5 + .../MATLAB Function ==
  data: yk_1 input; y_k output; uk_1 input; Pk_1 input; thetak_1 input; ek input; uk output; Pk output; theta_k output; t input; P output
function [y_k,uk,Pk,theta_k,P] = fcn(yk_1,uk_1,Pk_1,thetak_1,ek,t)
a=-0.8 - 0.1 * sin(0.1 * t);
b=0.5;
if t>=500
    b = 1;
end
P=[a;b];

if t>=0 && t<=50
    uk=0;
elseif t>=50 && t<51
    uk=1;
else
    uk=0;
end

sik=[-yk_1 uk_1]';
y_k=-a*yk_1+b*uk_1+ek;

Kk=Pk_1*sik*pinv(1+sik'*Pk_1*sik);
Pk=(eye(2,2)-Kk*sik')*Pk_1;
theta_k=thetak_1+Kk*(y_k-sik'*thetak_1);

== matlab function Q2_All/Q2_13/B/MATLAB Function ==
  data: yk_1 input; y_k output; uk_1 input; Pinvk_1 input; thetak_1 input; ek input; Pinvk output; theta_k output; P output; uk input; Uk output; ek_1 input; p11 output; p12 output; p13 output; p21 output; p22 output; p23 output; p31 output; p32 output; p33 output
function [y_k,Pinvk,theta_k,P,Uk,p11,p12,p13,p21,p22,p23,p31,p32,p33] = fcn(yk_1,uk_1,Pinvk_1,thetak_1,ek,uk,ek_1)
a=-0.8;
b=0.5;
c=-0.5;
P=[a;b;c];
Uk=uk;

sik=[-yk_1 uk_1 ek_1]';
y_k=-a*yk_1+b*uk_1+ek+c*ek_1;

Pinvk=Pinvk_1+sik*sik';
Pk=pinv(Pinvk);
epsilonk=y_k-sik'*thetak_1;
theta_k=thetak_1+Pk*sik*epsilonk;
p11=Pk(1,1);
p12=Pk(1,2);
p13=Pk(1,3);

p21=Pk(2,1);
p22=Pk(2,2);
p23=Pk(2,3);

p31=Pk(3,1);
p32=Pk(3,2);
p33=Pk(3,3);
